simulink model "Simulacion_PIL_NoIdeal"  (R2026a)
settings: Solver=VariableStepAuto  StopTime=2000  FixedStep=0.05  MaxStep=0.001
values from neighbouring files (symbols this model uses):
  den_s0 = G1 * G_eq    (= 0.172451295072)    [Modelado.m]
  den_s1 = (C_eq * G1) + (Cp * G1) + (Cp * G_eq)    (= 95.0203777143)    [Modelado.m]
  den_s2 = C_eq * Cp    (= 11224.6716568)    [Modelado.m]
  G1 = h1 * A1    (= 0.0428065366612)    [Modelado.m]
  num_Gamb = G_eq * [Cp, G1]    [Modelado.m]
libraries: sl_discontinuities x1
settings Model: Creator=magui  LastModifiedBy=Mariano M

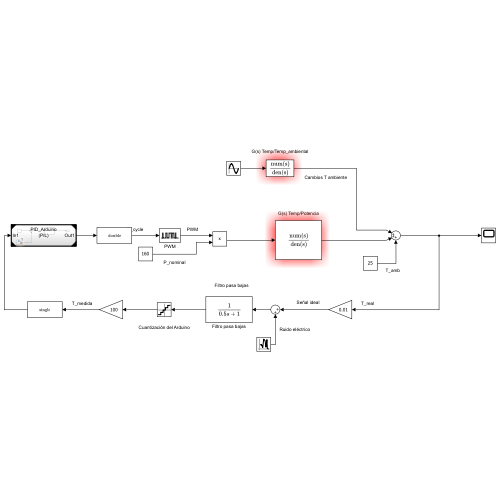
[thumbnail: Simulink's stored preview of the top-level diagram]
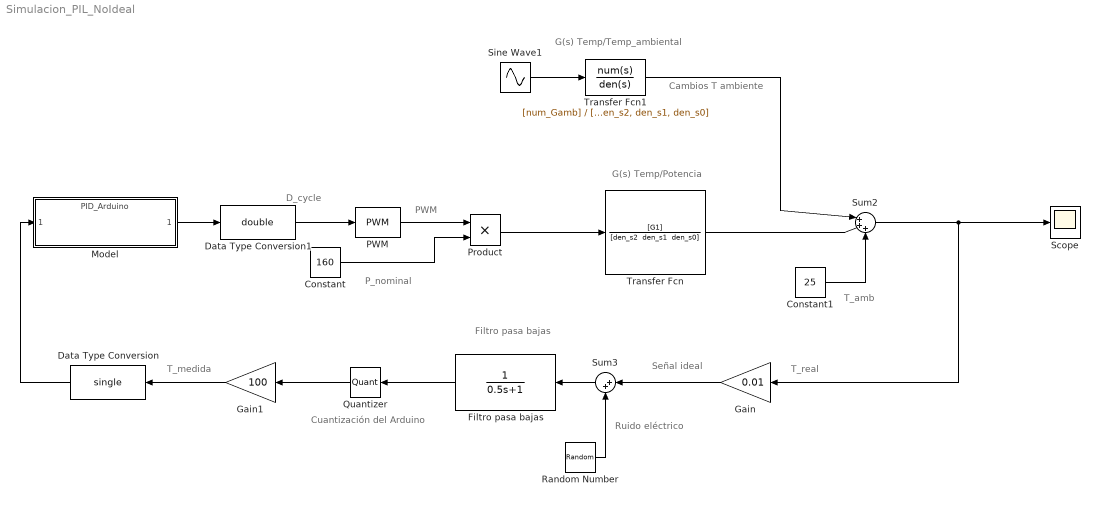
== system Simulacion_PIL_NoIdeal ==
  note: T_amb
  note: D_cycle
  note: T_real
  note: T_medida
  note: Ruido eléctrico
  note: Filtro pasa bajas
  note: Señal ideal
  note: Cambios T ambiente
  note: Cuantización del Arduino
  note: PWM
  note: P_nominal
  note: G(s) Temp/Potencia
  note: G(s) Temp/Temp_ambiental
  Constant : Constant  Value=160
  Constant1 : Constant  Value=25
  Data Type Conversion : DataTypeConversion  OutDataTypeStr=single  SaturateOnIntegerOverflow=off  RndMeth=Floor
  Data Type Conversion1 : DataTypeConversion  OutDataTypeStr=double  SaturateOnIntegerOverflow=off  RndMeth=Floor
  Filtro pasa bajas : TransferFcn  Denominator=[0.5 1]
  Gain : Gain  Gain=0.01
  Gain1 : Gain  Gain=100
  Model : ModelReference  ModelNameDialog=PID_Arduino.slx  SimulationMode=Processor-in-the-loop (PIL)  ModelReferenceVersion=1.15
  PWM : sl_discontinuities/PWM  DisableCoverage=on  Period=1/980  InitialDelay=0  DisallowZeroDutyCycle=off  RunAtFixedTimeIntervals=off  SampleTime=5e-5
      settings: LibrarySourceBlock=simulink/Discontinuities/PWM
  Product : Product
  Quantizer : Quantizer  QuantizationInterval=1.1/1024  LinearizeAsGain=off
  Random Number : RandomNumber  Variance=6.25e-6  Seed=1  SampleTime=0
  Scope : Scope
      settings: ActiveDisplayYMinimum=22.399201376206371  ActiveDisplayYMaximum=48.407187614142664
  Sine Wave1 : Sin  Amplitude=2  Frequency=6e-3  SampleTime=0
  Sum2 : Sum  Inputs=|+++
  Sum3 : Sum  Inputs=|++
  Transfer Fcn : TransferFcn  Numerator=[G1]  Denominator="[den_s2  den_s1  den_s0]"
  Transfer Fcn1 : TransferFcn  Numerator=[num_Gamb]  Denominator=[den_s2, den_s1, den_s0]
  wires:
  Gain/1 -> Sum3/1
  Transfer Fcn1/1 -> Sum2/1
  Random Number/1 -> Sum3/2
  Transfer Fcn/1 -> Sum2/2
  Sum2/1 -> Gain/1, Scope/1
  Constant1/1 -> Sum2/3
  Sum3/1 -> Filtro pasa bajas/1
  Filtro pasa bajas/1 -> Quantizer/1
  Quantizer/1 -> Gain1/1
  Product/1 -> Transfer Fcn/1
  Constant/1 -> Product/2
  Sine Wave1/1 -> Transfer Fcn1/1
  Model/1 -> Data Type Conversion1/1
  Gain1/1 -> Data Type Conversion/1
  Data Type Conversion/1 -> Model/1
  Data Type Conversion1/1 -> PWM/1
  PWM/1 -> Product/1
